simulink model "PID15m"  (Simulink 6.6)
settings: Solver=FixedStepDiscrete  StartTime=0.0  StopTime=.002  FixedStep=0.001  RelTol=1e-3
undefined symbols (not defined in the file or in its folder): QEIInit
libraries: dsPICdrivers x8, simulink x3, powerlib_extras x1
settings Model: Creator=123  LastModifiedBy=123  ProdHWDeviceType=16-bit Generic
settings OptimizationCC: OptimizeModelRefInitCode=on  LifeSpan=1
settings HardwareCC: ProdBitPerInt=16  ProdEndianess=LittleEndian  ProdWordSize=16  ProdHWDeviceType=16-bit Generic  TargetHWDeviceType=32-bit Generic
settings RTWCC: SystemTargetFile=dspic.tlc  TemplateMakefile=dspic_pic30_gcc.tmf  PostCodeGenCommand=dsPIC_Compile()  Description=Embedded Target for Microchip dsPIC (real-time)  ProcessScript=dspic_make_rtw_hook  CustomSource=myQEI.c
settings CodeAppCC: IgnoreCustomStorageClasses=off
settings STFCustomTargetCC: TargetFcnLib=ansi_tfl_tmw.mat  GenFloatMathFcnCalls=ANSI_C  ModelReferenceCompliant=off  IncludeMdlTerminateFcn=off  CombineOutputUpdateFcns=on  SuppressErrorStatus=on  ERTCustomFileBanners=on  SupportContinuousTime=off  SupportNonInlinedSFcns=off  SystemTargetFile=dspic.tlc
settings ERTTargetCC: TargetFcnLib=ansi_tfl_tmw.mat  GenFloatMathFcnCalls=ANSI_C  ModelReferenceCompliant=off  IncludeMdlTerminateFcn=off  SuppressErrorStatus=on  ModelStepFunctionPrototypeControlCompliant=off  InlinedParameterPlacement=NonHierarchical  ERTSrcFileBannerTemplate=dsPIC_code_template.cgt  ERTHdrFileBannerTemplate=dsPIC_code_template.cgt  ERTDataSrcFileTemplate=dsPIC_code_template.cgt  ERTDataHdrFileTemplate=dsPIC_code_template.cgt  ERTCustomFileTemplate=dsPIC_main.tlc
settings CustomProperty: DataType=string  Value=C:\PROGRA~2\MATLAB\R2007a\rtw\bin\win32\gmake

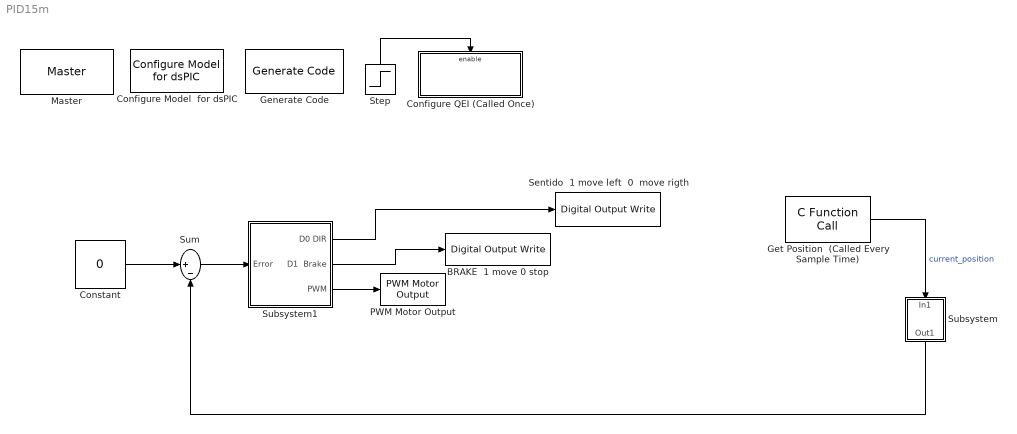
== system PID15m ==
  BRAKE  1 move 0 stop : dsPICdrivers/Digital I//O/Digital Output Write  Tag=dsPIC_Digital_Output  Priority=5  PORT=D  Pin=[1]  Simultaneous=off  OrderingInOutPopup=None
  Configure Model  for dsPIC : dsPICdrivers/Simulink Configuration/Configure Model  for dsPIC
  Configure QEI (Called Once) : Subsystem  TreatAsAtomicUnit=on
  Constant : Constant  Value=0  OutDataTypeMode=int32  SampleTime=.001
  Generate Code : dsPICdrivers/Simulink Configuration/Generate Code
  Get Position  (Called Every Sample Time) : dsPICdrivers/OTHERS/C Function Call  Tag=dsPIC_dsPIC_CFunctionCall  fctName='GetQEI'  INPUT_SIZE=1  INPUT1=--  INPUT2=--  INPUT3=--  OUTPUT_SIZE=1  OUTPUT1=int32  SampleTime=.001  InputType=[ ]  OutputType=[ 5 ]  FctDeclaration=extern int32_T GetQEI();  FctCall=%y1 = GetQEI();  OrderingInOutPopup=None
  Master : dsPICdrivers/Master  Tag=dsPIC_MASTER  Priority=1  TimeStepType=Timer1  picType=30f4012  fcy=30e6  Quartz_33f=5e6  PLLActive_33f=off  fcyDesired_33f=0  tmr1="[1  29999  0]"  tmr1Info="Time Step : 0.001  ;   Error : 0%  PR1=29999"  tmr2345="[0  0  0  0]"  tmr2345cfg=[-1 -1 -1 -1]  IOautoConf=on  typePort="[ 0   0   0   0   0   0   0   0   0   0   0   0   0   0   0   0   0   0   0   0   0   0   0   0   0   0   0   0   0   0   0   0   0   0   0   0   0   0   0   0   0   0   0   0   0   0   0   0  10  10   0   0   0   0   0   0   0   0   0   0   0   0   0   0  11   0   0   0   0   0   0   0   0   0   0   0   0   0   0   0   0   0   0   0   0   0   0   0   0   0   0   0   0   0   0   0   0   0   0   0   0   0   0   0   0   0   0   0   0   0   0   0 ]"  TRIS="[ 65535  65535  65535  65532  65535  65535  65535 ]"  ADPCFG=0  MasterBusyPort=None  MasterOverloadPort=None  FOSC=FRC_PLL16  ClockSwitchMonitor=Both disabled  TempProtection_33f=TEMP_ON  FPBOR=PBOR_OFF  PWRT=PWRT_OFF  MCLR=MCLR_DIS  PowerSave=off  OverrideFcy=off  NewFcy=1e6
  PWM Motor Output : dsPICdrivers/Peripheral I//O/PWM Motor Output  Tag=dsPIC_PWM_Motor  Priority=5  InputEnableChk=off  InputPeriodeChk=off  Channel=[1 ]  TPeriode=.01  PrescalerValue=16  PeriodeInteger=18750  MaxName='PWM'  Centered=off  HChannelON=off  Info="Nbr Bits : 15.1946  ||  PWM = 37500  ||  Prescaler = 16"  Delay=0  IntPriority=5  nbrPwmChannelPIC=3  Status=OK
  Sentido  1 move left  0  move rigth : dsPICdrivers/Digital I//O/Digital Output Write  Tag=dsPIC_Digital_Output  Priority=5  PORT=D  Pin=[0]  Simultaneous=off  OrderingInOutPopup=None
  Step : Step  Orientation=up  Time=0.002  Before=1  After=0  SampleTime=0.001
  Subsystem : Subsystem  Orientation=down
  Subsystem1 : Subsystem
  Sum : Sum  Inputs=|+-
  wires:
  Step/1 -> Configure QEI (Called Once)/Enable
  Get Position  (Called Every Sample Time)/1 -> Subsystem/1(In1)  "current_position"
  Subsystem/1(Out1) -> Sum/2
  Sum/1 -> Subsystem1/1(Error)
  Subsystem1/1(D0 DIR) -> Sentido  1 move left  0  move rigth/1
  Subsystem1/3(PWM) -> PWM Motor Output/1
  Subsystem1/2(D1  Brake) -> BRAKE  1 move 0 stop/1
  Constant/1 -> Sum/1

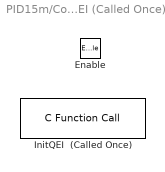
== system PID15m/Configure QEI (Called Once) ==
  Enable : EnablePort
  InitQEI  (Called Once) : dsPICdrivers/OTHERS/C Function Call  Tag=dsPIC_dsPIC_CFunctionCall  fctName='QEIInit'  INPUT_SIZE=1  INPUT1=--  INPUT2=--  INPUT3=--  OUTPUT_SIZE=1  OUTPUT1=--  SampleTime=inf  InputType=[ ]  OutputType=[ ]  FctDeclaration=extern void QEIInit();  FctCall=QEIInit();  OrderingInOutPopup=None

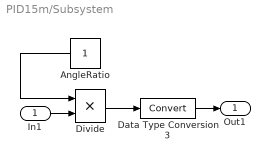
== system PID15m/Subsystem ==
  In1 : Inport
  AngleRatio : Constant  Orientation=left  SampleTime=.001
  Data Type Conversion3 : DataTypeConversion  OutDataTypeMode=int32  SampleTime=.001
  Divide : Product  Inputs=**  OutScaling=2^-10  SampleTime=.001
  Out1 : Outport
  wires:
  AngleRatio/1 -> Divide/1
  Divide/1 -> Data Type Conversion3/1
  Data Type Conversion3/1 -> Out1/1
  In1/1 -> Divide/2

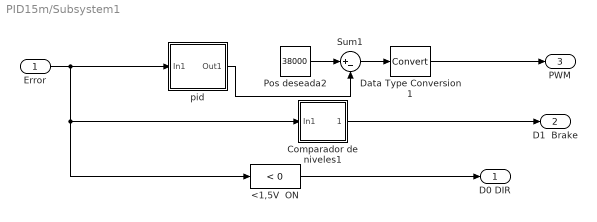
== system PID15m/Subsystem1 ==
  Error : Inport
  <1,5V  ON : simulink/Logic and Bit Operations/Compare To Constant  SystemSampleTime=-1  relop=<  const=0  LogicOutDataTypeMode=boolean  ZeroCross=off
  Comparador de niveles1 : Subsystem
  Data Type Conversion1 : DataTypeConversion  OutDataTypeMode=uint16  SampleTime=.001
  Pos deseada2 : Constant  Value=38000  SampleTime=.001
  Sum1 : Sum  Inputs=|+-  SampleTime=.001
  pid : Subsystem
  D0 DIR : Outport
  D1  Brake : Outport  Port=2
  PWM : Outport  Port=3
  wires:
  Error/1 -> pid/1(In1), <1,5V  ON/1, Comparador de niveles1/1(In1)
  Pos deseada2/1 -> Sum1/1
  pid/1(Out1) -> Sum1/2
  Sum1/1 -> Data Type Conversion1/1
  Data Type Conversion1/1 -> PWM/1
  Comparador de niveles1/1(Out1) -> D1  Brake/1
  <1,5V  ON/1 -> D0 DIR/1

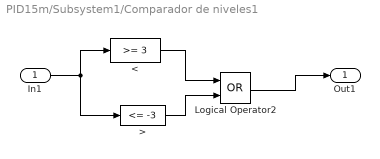
== system PID15m/Subsystem1/Comparador de niveles1 ==
  In1 : Inport
  < : simulink/Logic and Bit Operations/Compare To Constant  SystemSampleTime=-1  relop=>=  const=3  LogicOutDataTypeMode=boolean  ZeroCross=off
  "> " : simulink/Logic and Bit Operations/Compare To Constant  SystemSampleTime=-1  relop=<=  const=-3  LogicOutDataTypeMode=boolean  ZeroCross=off
  Logical Operator2 : Logic  Operator=OR  AllPortsSameDT=off  OutDataTypeMode=Boolean  SampleTime=.001
  Out1 : Outport
  wires:
  </1 -> Logical Operator2/1
  "> "/1 -> Logical Operator2/2
  In1/1 -> "> "/1, </1
  Logical Operator2/1 -> Out1/1

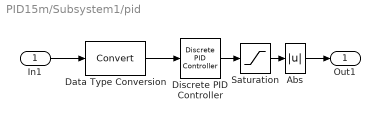
== system PID15m/Subsystem1/pid ==
  In1 : Inport
  Abs : Abs  SampleTime=.001
  Data Type Conversion : DataTypeConversion  SampleTime=.001
  Discrete PID Controller : powerlib_extras/Discrete  Control Blocks/Discrete PID Controller  DialogController=POWERSYS.PowerSysDialog  SystemSampleTime=-1  Kp=40  Ki=0.1  Kd=.3  TcD=0.5e-3  Par_Limits=[1e6 -1e6]  Init=0  Ts=.001
  Saturation : Saturate  UpperLimit=38000  LowerLimit=-38000  SampleTime=.001
  Out1 : Outport
  wires:
  Discrete PID Controller/1 -> Saturation/1
  Data Type Conversion/1 -> Discrete PID Controller/1
  Saturation/1 -> Abs/1
  In1/1 -> Data Type Conversion/1
  Abs/1 -> Out1/1
